simulink model "MCC"  (R2021b)
settings: Solver=ode1  StartTime=0.0  StopTime=10  FixedStep=1e-5  RelTol=1e-3
libraries: spsSeriesRLCBranchLib x2, spsControlledVoltageSourceLib x1, spsCurrentMeasurementLib x1, spsDCVoltageSourceLib x1, spsDiodeLib x1, spsDCMachineLib x1, spsMosfetLib x1, spsVoltageMeasurementLib x1, spspowerguiLib x1
settings Model: Creator=Guo Qihao  LastModifiedBy=szenia
settings SolverCC: AlgebraicLoopSolver=TrustRegion
settings DebuggingCC: SFMachineParentedDataDiag=warning  ArithmeticOperatorsInVariantConditions=warning
settings SFSimCC: CustomCodeUndefinedFunction=UseInterfaceOnly

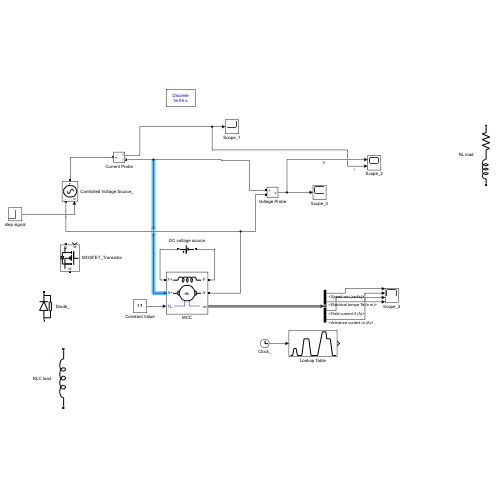
[thumbnail: Simulink's stored preview of the top-level diagram]
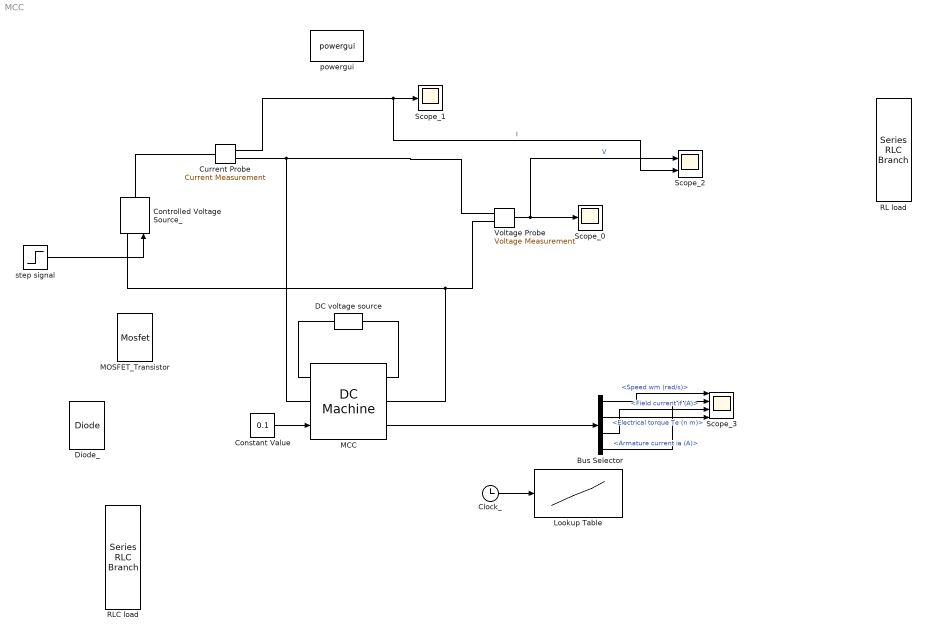
== system MCC ==
  Bus Selector : BusSelector  OutputSignals=Speed wm (rad/s),Electrical torque Te (n m),Field current if (A),Armature current ia (A)
  Clock_ : Clock
  Constant Value : Constant  Value=0.1
  Controlled Voltage Source_ : spsControlledVoltageSourceLib/Controlled Voltage Source  Initialize=off  Source_Type=DC  Amplitude=0  Phase=0  Frequency=0  Measurements=None
  Current Probe : spsCurrentMeasurementLib/Current Measurement  PhasorSimulation=off  OutputType=Complex  PSBequivalent=0
  DC voltage source : spsDCVoltageSourceLib/DC Voltage Source  Amplitude=200  Measurements=None
  Diode_ : spsDiodeLib/Diode  Ron=0.001  Lon=0  Vf=0.8  IC=0  UseSnubber=off  Rs=500  Cs=250e-9  Measurements=off
  Lookup Table : Lookup  InputValues=[0,10,15,25,30,50,60,80,90,120,140,155,160,175,185,200]  Table=[0,0,15,15,0,0,35,35,0,0,50,50,35,35,0,0]
  MCC : spsDCMachineLib/DC Machine  PresetModel=No  MechanicalLoad=Torque TL  FieldType=Wound  ShowDetailedParameters=on  MeasurementBus=off  RLa=[1.5 0.01]  RLf=[ 7 0.09]  Laf=0.01  MachineConstant=Torque constant (N.m/A)  Ke=1.8  Kt=1.8  J=0.1  Bm=0  Tf=0  w0=1  Ifinit=0  TsPowergui=0  TsBlock=-1
  MOSFET_Transistor : spsMosfetLib/Mosfet  Ron=0.004  Lon=0  Rd=0.01  Vfd=0  IC=0  Rs=1e5  Cs=inf  Measurements=off
  RL load : spsSeriesRLCBranchLib/Series RLC Branch  LConnTagsString=__new0  RConnTagsString=__new0  BranchType=RL  Resistance=1  Inductance=1e-2  SetiL0=off  InitialCurrent=0  Capacitance=0  Setx0=off  InitialVoltage=0  Measurements=Branch current
  RLC load : spsSeriesRLCBranchLib/Series RLC Branch  LConnTagsString=__new0  RConnTagsString=__new0  BranchType=L  Resistance=1  Inductance=1e-2  SetiL0=off  InitialCurrent=0  Capacitance=0  Setx0=off  InitialVoltage=0  Measurements=Branch current
  Scope_0 : Scope
  Scope_1 : Scope
  Scope_2 : Scope  NumInputPorts=2
  Scope_3 : Scope  NumInputPorts=4
  Voltage Probe : spsVoltageMeasurementLib/Voltage Measurement  PhasorSimulation=off  OutputType=Complex  PSBequivalent=0
  powergui : spspowerguiLib/powergui  Priority=1  SimulationMode=Discrete  SampleTime=1e-5  frequency=60  Iterations=50  frequencyindice=0  Pbase=100e6  ErrMax=1e-4  UnitsV=kV  UnitsW=MW  buscounter=0  FunctionMessages=off  echomessages=off  EnableUseOfTLC=off  CurrentSourceSwitches=off  DisableSnubberDevices=off  DisableRonSwitches=off  DisableVfSwitches=off  DisplayEquations=off  AutomaticDiscreteSolvers=off  SolverType=Tustin/Backward Euler (TBE)  Interpol=off  ExternalGateDelay=off  methode=off  Ts=100  x0status=zero  SPID=on  SwTol=0  HookPort=off  NonlinearTolerance=1e-4  nMaxIteration=100  ContinueOnMaxIteration=off  RestoreLinks=warning  ResistiveCurrentMeasurement=off  Frange=[0:2:500]  Ylog=off  Xlog=on  ShowGrid=off  save=off  variable=ZData  structure=0  ZoomFFT=off  StartTime=0.0  cycles=1  DisplayStyle=1  fundamental=60  FreqAxis=off  MaxFrequency=1000  frequencyindicesteady=1  RmsSteady=1  display=off
  step signal : Step  Time=0.5  Before=1  After=120  SampleTime=0
  wires:
  Current Probe/1 -> Scope_2/2, Scope_1/1  "I"
  step signal/1 -> Controlled Voltage Source_/1
  Voltage Probe/1 -> Scope_2/1, Scope_0/1  "V"
  Clock_/1 -> Lookup Table/1
  MCC/1 -> Bus Selector/1
  Constant Value/1 -> MCC/1
  Bus Selector/1 -> Scope_3/1  "<Speed wm (rad/s)>"
  Bus Selector/2 -> Scope_3/4  "<Electrical torque Te (n m)>"
  Bus Selector/3 -> Scope_3/3  "<Field current if (A)>"
  Bus Selector/4 -> Scope_3/2  "<Armature current ia (A)>"
  connections:
  Current Probe/LConn1 -- Controlled Voltage Source_/RConn1
  Voltage Probe/LConn1 -- Current Probe/RConn1 -- MCC/LConn1
  Voltage Probe/LConn2 -- MCC/RConn1 -- Controlled Voltage Source_/LConn1
  DC voltage source/RConn1 -- MCC/LConn2
  DC voltage source/LConn1 -- MCC/RConn2
